simulink model "Controller_kinesthetic_01"  (R2026b)
settings: Solver=ode4  StopTime=Inf  FixedStep=1e-3
values from neighbouring files (symbols this model uses):
  Dn = 20*ones(7,1)    [Controller_taskSpace_Init.m]
  H_0_cy = H_0_pr*H_pr_cy    [Controller_taskSpace_Init.m]
  H_home = getTransform(Franka_robot, q_home, 'panda_link8','panda_link0')    [Controller_taskSpace_Init.m]
  Kn = 20*ones(7,1)    [Controller_taskSpace_Init.m]
  q_home = [0.003542735427650;-0.076954344513307;-0.003006835131443;-1.362053944077202;-5.624494697578509e-04;1.279919277568267;0.786445509714290]    [Controller_taskSpace_Init.m]
  q_init = alpha_3.*s^3 + alpha_2.*s^2 + alpha_1.*s + alpha_0    [Controller_taskSpace_Init.m]
  s = 0    [Controller_taskSpace_Init.m]
undefined symbols (not defined in the file or in its folder): DiscIntNeverNeededParam, Fext_mag, T_final, X, Y, Z
libraries: sm_lib x162, nesl_utility x44, matrix_library x3, Robotics_lib x1
(part 11 of 11)

== matlab function Controller_kinesthetic_01/task space controller/MATLAB Function2 ==
  data: H_IT input; x_c output size=1; v_c output size=1; V_tilde input; lambda_mat input; n_hp input; m_c output size=1; xTableHight input; eef_height input
function [x_c, v_c, m_c] = fcn(H_IT, V_tilde, lambda_mat, n_hp, xTableHight, eef_height)

auxMat = zeros(4,4);
auxMat(3,4) = -xTableHight;

H = H_IT*[eye(3), [0;0;eef_height];zeros(1,3),1] + auxMat;

x_c = transpose(n_hp)*[H(1:3,4);zeros(3,1)];

v_c = transpose(n_hp)*V_tilde;




lambda_inv = lambda_mat\eye(6);
lambda_inv = (lambda_inv + transpose(lambda_inv))./2;

tmp3 = transpose(n_hp)*lambda_inv*n_hp;
m_c = tmp3\eye(1);


end

== matlab function Controller_kinesthetic_01/Dynamic Parameters/End Effector ==
  data: q input; H_0e output
function H_0e = H_0e(q)
% Author: TU Wien, ACIN Robotics group
% Optimized and generated from Maple
  H_0e = zeros(4,4);
  t4449 = q(6);
  t4435 = sin(t4449);
  t4442 = cos(t4449);
  t4431 = 0.107e0 * t4435 + 0.88e-1 * t4442;
  t4450 = q(5);
  t4436 = sin(t4450);
  t4452 = q(3);
  t4438 = sin(t4452);
  t4491 = t4438 * t4436;
  t4499 = t4431 * t4491;
  t4430 = 0.107e0 * t4442 - 0.88e-1 * t4435 - 0.384e0;
  t4451 = q(4);
  t4437 = sin(t4451);
  t4498 = -t4430 * t4437 - 0.825e-1;
  t4443 = cos(t4450);
  t4427 = t4431 * t4443 - 0.825e-1;
  t4444 = cos(t4451);
  t4497 = t4427 * t4444;
  t4495 = t4430 * t4444;
  t4448 = q(7);
  t4434 = sin(t4448);
  t4454 = q(1);
  t4440 = sin(t4454);
  t4494 = t4434 * t4440;
  t4493 = t4436 * t4437;
  t4492 = t4437 * t4435;
  t4490 = t4438 * t4442;
  t4489 = t4438 * t4443;
  t4441 = cos(t4448);
  t4488 = t4440 * t4441;
  t4487 = t4443 * t4437;
  t4486 = t4443 * t4444;
  t4445 = cos(t4452);
  t4485 = t4443 * t4445;
  t4484 = t4444 * t4435;
  t4483 = t4445 * t4436;
  t4482 = t4445 * t4437;
  t4481 = t4445 * t4444;
  t4453 = q(2);
  t4439 = sin(t4453);
  t4446 = cos(t4453);
  t4467 = t4436 * t4481;
  t4458 = (t4467 + t4489) * t4446;
  t4478 = t4434 * t4493;
  t4480 = t4434 * t4458 + t4439 * t4478;
  t4479 = t4431 * t4483;
  t4477 = t4442 * t4487;
  t4476 = t4436 * t4490;
  t4475 = t4444 * t4491;
  t4474 = t4441 * t4493;
  t4473 = t4437 * t4490;
  t4472 = t4442 * t4486;
  t4471 = t4442 * t4483;
  t4470 = t4440 * t4485;
  t4469 = t4438 * t4486;
  t4468 = t4443 * t4481;
  t4466 = t4427 * t4437 + 0.316e0;
  t4465 = t4497 - t4498;
  t4464 = -0.1e1 * t4497 + t4498;
  t4463 = t4477 + t4484;
  t4462 = t4472 - 0.1e1 * t4492;
  t4461 = -0.1e1 * t4472 + t4492;
  t4460 = -0.1e1 * t4477 - 0.1e1 * t4484;
  t4459 = -0.1e1 * t4467 - 0.1e1 * t4489;
  t4447 = cos(t4454);
  t4457 = (t4475 - 0.1e1 * t4485) * t4447;
  t4456 = t4438 * t4462 + t4471;
  t4455 = -0.1e1 * t4471 + t4461 * t4438;
  t4425 = t4445 * t4461 + t4476;
  t4424 = t4462 * t4445 - 0.1e1 * t4476;
  t4423 = ((-0.1e1 * t4491 + t4468) * t4446 + t4439 * t4487) * t4435 + (t4446 * t4482 - 0.1e1 * t4439 * t4444) * t4442;
  t4422 = t4424 * t4446 + t4439 * t4463;
  t4421 = (t4425 * t4446 + t4439 * t4460) * t4434 + t4441 * t4458 + t4439 * t4474;
  t4420 = (t4465 * t4445 - 0.1e1 * t4499) * t4446 + (-0.1e1 * t4495 + t4466) * t4439;
  H_0e(1,3) = t4423 * t4447 + ((-0.1e1 * t4483 - 0.1e1 * t4469) * t4435 - 0.1e1 * t4473) * t4440;
  H_0e(4,1) = 0.0e0;
  H_0e(4,3) = 0.0e0;
  H_0e(3,1) = (t4425 * t4439 + t4446 * t4463) * t4441 + t4459 * t4434 * t4439 + t4446 * t4478;
  H_0e(2,1) = (t4422 * t4440 + t4447 * t4456) * t4441 + t4480 * t4440 + t4434 * t4457;
  H_0e(4,4) = 0.1e1;
  H_0e(3,2) = (t4424 * t4434 + t4441 * t4459) * t4439 + (t4434 * t4460 + t4474) * t4446;
  H_0e(3,4) = (t4445 * t4464 + t4499) * t4439 + 0.333e0 + (t4466 - t4495) * t4446;
  H_0e(2,3) = t4423 * t4440 + ((t4469 + t4483) * t4435 + t4473) * t4447;
  H_0e(2,4) = t4420 * t4440 + (t4438 * t4465 + t4479) * t4447;
  H_0e(4,2) = 0.0e0;
  H_0e(2,2) = t4434 * t4447 * t4455 + t4421 * t4440 + t4441 * t4457;
  H_0e(1,1) = (t4422 * t4441 + t4480) * t4447 + t4455 * t4488 - 0.1e1 * t4475 * t4494 + t4434 * t4470;
  H_0e(3,3) = ((t4491 - 0.1e1 * t4468) * t4435 - 0.1e1 * t4442 * t4482) * t4439 + (-0.1e1 * t4442 * t4444 + t4435 * t4487) * t4446;
  H_0e(1,4) = t4420 * t4447 + (-0.1e1 * t4479 + t4464 * t4438) * t4440;
  H_0e(1,2) = t4421 * t4447 + t4456 * t4494 - 0.1e1 * t4475 * t4488 + t4441 * t4470;
end
